simulink subsystem "multimodecbf_subsystem"  (R2025b)
settings: Solver=VariableStepAuto  StartTime=0.0  StopTime=10.0  RelTol=1e-3
settings Model: Creator=sanborkl  LastModifiedBy=sanborkl

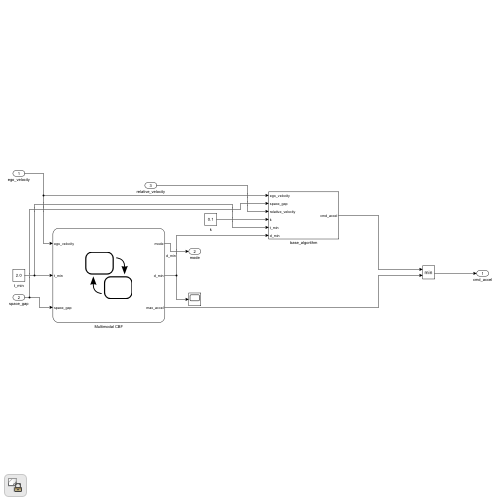
[thumbnail: Simulink's stored preview of the top-level diagram]
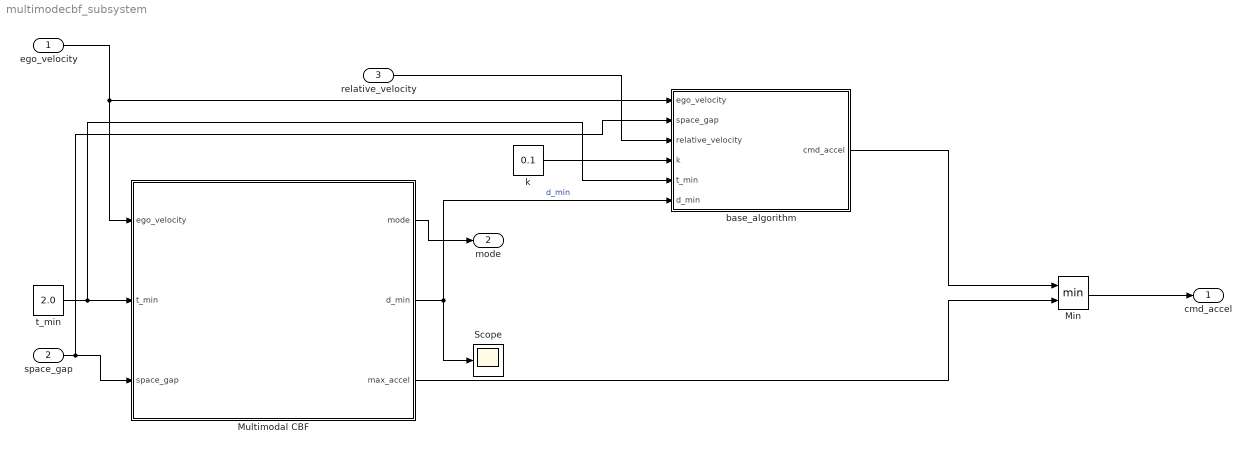
== system multimodecbf_subsystem ==
  ego_velocity : Inport
  space_gap : Inport  Port=2
  relative_velocity : Inport  Port=3
  Min : MinMax  Inputs=2
  Multimodal CBF : Stateflow chart  TreatAsAtomicUnit=on
  Scope : Scope
      settings: ActiveDisplayYMinimum=3.7500000000000004  ActiveDisplayYMaximum=16.25  DataLoggingVariableName=ScopeData12
  base_algorithm : Subsystem
  k : Constant  Value=0.1
  t_min : Constant  Value=2.0
  cmd_accel : Outport
  mode : Outport  Port=2
  wires:
  relative_velocity/1 -> base_algorithm/3(relative_velocity)
  Min/1 -> cmd_accel/1
  ego_velocity/1 -> base_algorithm/1(ego_velocity), Multimodal CBF/1(ego_velocity)
  t_min/1 -> base_algorithm/5(t_min), Multimodal CBF/2(t_min)
  Multimodal CBF/3(max_accel) -> Min/2
  space_gap/1 -> base_algorithm/2(space_gap), Multimodal CBF/3(space_gap)
  Multimodal CBF/2(d_min) -> base_algorithm/6(d_min), Scope/1  "d_min"
  base_algorithm/1(cmd_accel) -> Min/1
  Multimodal CBF/1(mode) -> mode/1
  k/1 -> base_algorithm/4(k)

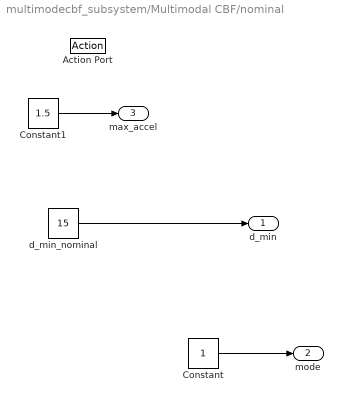
== system multimodecbf_subsystem/Multimodal CBF/nominal ==
  Action Port : ActionPort
      settings: CopyFcn=Stateflow.SLINSF.SimulinkMan.removeBlockPreDeleteFcn  PreDeleteFcn=Stateflow.SLINSF.SimulinkMan.unsafePredeleteFcn
  Constant : Constant
  Constant1 : Constant  Value=1.5
  d_min_nominal : Constant  Value=15
  d_min : Outport
  mode : Outport  Port=2
  max_accel : Outport  Port=3
  wires:
  Constant/1 -> mode/1
  d_min_nominal/1 -> d_min/1
  Constant1/1 -> max_accel/1

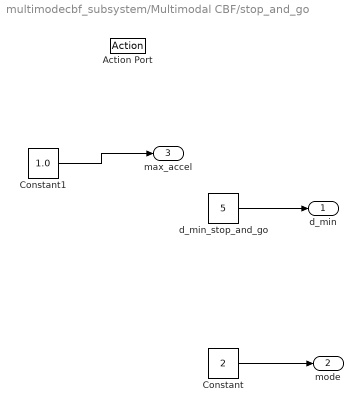
== system multimodecbf_subsystem/Multimodal CBF/stop_and_go ==
  Action Port : ActionPort
      settings: CopyFcn=Stateflow.SLINSF.SimulinkMan.removeBlockPreDeleteFcn  PreDeleteFcn=Stateflow.SLINSF.SimulinkMan.unsafePredeleteFcn
  Constant : Constant  Value=2
  Constant1 : Constant  Value=1.0
  d_min_stop_and_go : Constant  Value=5
  d_min : Outport
  mode : Outport  Port=2
  max_accel : Outport  Port=3
  wires:
  d_min_stop_and_go/1 -> d_min/1
  Constant/1 -> mode/1
  Constant1/1 -> max_accel/1

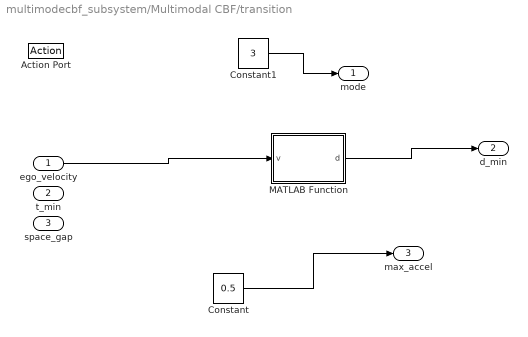
== system multimodecbf_subsystem/Multimodal CBF/transition ==
  ego_velocity : Inport
  t_min : Inport  Port=2
  space_gap : Inport  Port=3
  Action Port : ActionPort
      settings: CopyFcn=Stateflow.SLINSF.SimulinkMan.removeBlockPreDeleteFcn  PreDeleteFcn=Stateflow.SLINSF.SimulinkMan.unsafePredeleteFcn
  Constant : Constant  Value=0.5
  Constant1 : Constant  Value=3
  MATLAB Function : MATLAB Function  TreatAsAtomicUnit=on
  mode : Outport
  d_min : Outport  Port=2
  max_accel : Outport  Port=3
  wires:
  Constant/1 -> max_accel/1
  Constant1/1 -> mode/1
  MATLAB Function/1(d) -> d_min/1
  ego_velocity/1 -> MATLAB Function/1(v)

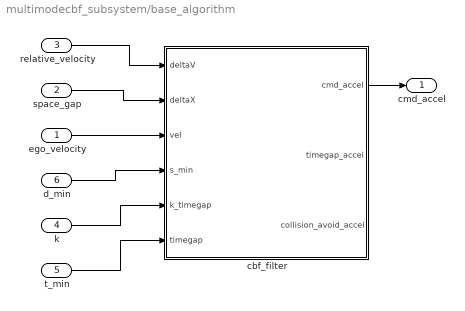
== system multimodecbf_subsystem/base_algorithm ==
  ego_velocity : Inport
  space_gap : Inport  Port=2
  relative_velocity : Inport  Port=3
  k : Inport  Port=4
  t_min : Inport  Port=5
  d_min : Inport  Port=6
  cbf_filter : Subsystem
  cmd_accel : Outport
  wires:
  space_gap/1 -> cbf_filter/2(deltaX)
  k/1 -> cbf_filter/5(k_timegap)
  cbf_filter/1(cmd_accel) -> cmd_accel/1
  d_min/1 -> cbf_filter/4(s_min)
  ego_velocity/1 -> cbf_filter/3(vel)
  t_min/1 -> cbf_filter/6(timegap)
  relative_velocity/1 -> cbf_filter/1(deltaV)

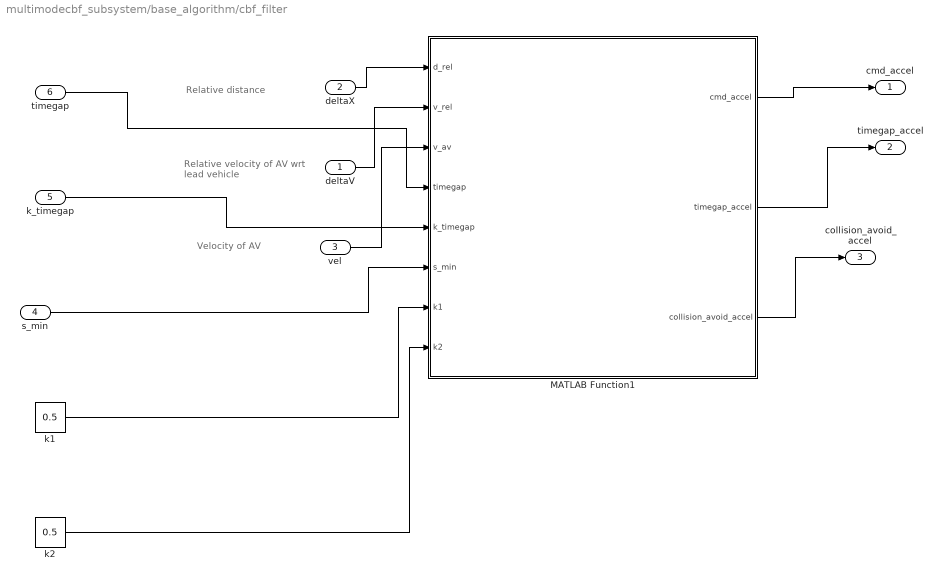
== system multimodecbf_subsystem/base_algorithm/cbf_filter ==
  note: Relative distance
  note: Relative velocity of
      | AV wrt lead vehicle
  note: Velocity of AV
  deltaV : Inport
  deltaX : Inport  Port=2
  vel : Inport  Port=3
  s_min : Inport  Port=4
  k_timegap : Inport  Port=5
  timegap : Inport  Port=6
  MATLAB Function1 : MATLAB Function  TreatAsAtomicUnit=on
  k1 : Constant  Value=0.5
  k2 : Constant  Value=0.5
  cmd_accel : Outport
  timegap_accel : Outport  Port=2
  collision_avoid_accel : Outport  Port=3
  wires:
  MATLAB Function1/3(collision_avoid_accel) -> collision_avoid_accel/1
  k2/1 -> MATLAB Function1/8(k2)
  deltaX/1 -> MATLAB Function1/1(d_rel)
  deltaV/1 -> MATLAB Function1/2(v_rel)
  vel/1 -> MATLAB Function1/3(v_av)
  MATLAB Function1/1(cmd_accel) -> cmd_accel/1
  MATLAB Function1/2(timegap_accel) -> timegap_accel/1
  s_min/1 -> MATLAB Function1/6(s_min)
  k_timegap/1 -> MATLAB Function1/5(k_timegap)
  timegap/1 -> MATLAB Function1/4(timegap)
  k1/1 -> MATLAB Function1/7(k1)

== matlab function multimodecbf_subsystem/base_algorithm/cbf_filter/MATLAB Function1 ==
  data: cmd_accel output; d_rel input; v_rel input; v_av input; timegap input; timegap_accel output; collision_avoid_accel output; k_timegap input; s_min input; k1 input; k2 input
function [cmd_accel, timegap_accel, collision_avoid_accel]= fcn(d_rel,v_rel,v_av, timegap,k_timegap,s_min,k1,k2)
%#codegen

% from the timegap filter function
% maybe make this gain a parameter later
% k = 0.1;
k = k_timegap;
%t_min = 2.0;
t_min = timegap;
timegap_accel = (1/t_min)*v_rel + (k/t_min)*(d_rel - t_min*v_av - s_min);

% from collision-avoid filter function
% a potential parameter - read into the fcn now
% s_min = 15.0;
% a potential parameter - read into the fcn now
% k1 = 0.5;
% a potential parameter - read into the fcn now
% k2 = 0.5;
%a_max = a_l + (k1+k2)*(delta_v) + (k1*k2)*(s-s_min);
% simplification TODO this is maybe dangerous so need to confirm
a_l = 0;
collision_avoid_accel = a_l + (k1+k2)*(v_rel) + (k1*k2)*(d_rel-s_min);

% now put these together
% 	 tg_accel = time_gap_filter(v,s,delta_v)
% 	 ca_accel = collision_avoid_filter(s,delta_v,a_l)
% 	 return min([tg_accel,ca_accel])
% TODO make max/min acceleration parameters.
% cmd_accel = min(1.5,max(-3.0,min(timegap_accel,collision_avoid_accel)));

% cmd_accel = min(timegap_accel,collision_avoid_accel);
cmd_accel = timegap_accel;

== stateflow chart multimodecbf_subsystem/Multimodal CBF ==
  state transition
  state stop_and_go
  state nominal
  stop_and_go -> transition : [(ego_velocity >= 7.5) & (space_gap >= t_min * ego_velocity + 5 - 0.1)]
  transition -> nominal [order 2] : [(space_gap >= t_min * ego_velocity + 15 - 0.1) & (ego_velocity > 5)]
  transition -> stop_and_go [order 1] : [ego_velocity <= 5]
  (default) -> nominal : {d_min=15; mode=1; max_accel=1.5;}
  nominal -> stop_and_go : [(space_gap >= t_min * ego_velocity + 15 - 0.1) & duration(ego_velocity <= 5, 'sec') >= 3]
  data: sf_internal_action_state_placeholder_data local double size=1 =0; sf_internal_action_state_placeholder_data local double size=1 =0; sf_internal_action_state_placeholder_data local double size=1 =0; ego_velocity input; mode output; d_min output; t_min input; space_gap input; max_accel output

== matlab function multimodecbf_subsystem/Multimodal CBF/transition/MATLAB Function ==
  data: v input; d output
function d = fcn(v)

e_term = exp(3.0 * (v - 6.25));

fraction = e_term / (1 + e_term);

d = 10 * fraction + 5;
